simulink model "RC_protect"  (Simulink 6.4)
settings: Solver=FixedStepDiscrete  StartTime=0.0  StopTime=10.0  FixedStep=0.001  RelTol=1e-3
libraries: dsPICdrivers x4, simulink x1
CloseFcn:
  | rtwprivate ssgencode ModelCloseRequest dspic_sensorless
settings Model: DataTypeOverride=ForceOff  MinMaxOverflowLogging=ForceOff  Creator=Lubin  LastModifiedBy=lubink
settings OptimizationCC: InlineParams=on  InlineInvariantSignals=on  EnforceIntegerDowncast=off  StateBitsets=on  DataBitsets=on  UseTempVars=on  ZeroExternalMemoryAtStartup=off  ZeroInternalMemoryAtStartup=off  InitFltsAndDblsToZero=off  OptimizeModelRefInitCode=on  LifeSpan=1
settings DebuggingCC: MultiTaskDSMMsg=error  MultiTaskCondExecSysMsg=error
settings HardwareCC: ProdBitPerInt=16  ProdEndianess=LittleEndian  ProdWordSize=16  ProdHWDeviceType=16-bit Generic  TargetHWDeviceType=32-bit Generic
settings RTWCC: SystemTargetFile=dspic.tlc  TemplateMakefile=dspic_pic30_gcc.tmf  PostCodeGenCommand=dsPIC_Compile()  Description=Embedded Target for Microchip dsPIC (real-time)  GenerateReport=on  ProcessScript=dspic_make_rtw_hook  IncludeHyperlinkInReport=on  LaunchReport=on
settings CodeAppCC: IgnoreCustomStorageClasses=off
settings STFCustomTargetCC: TargetFcnLib=ansi_tfl_tmw.mat  GenFloatMathFcnCalls=ANSI_C  ModelReferenceCompliant=off  IncludeMdlTerminateFcn=off  CombineOutputUpdateFcns=on  SuppressErrorStatus=on  ERTCustomFileBanners=on  SupportContinuousTime=off  SupportNonInlinedSFcns=off  ModelStepFunctionPrototypeControlCompliant=on  SystemTargetFile=dspic.tlc
settings ERTTargetCC: TargetFcnLib=ansi_tfl_tmw.mat  GenFloatMathFcnCalls=ANSI_C  ModelReferenceCompliant=off  ParMdlRefBuildCompliant=off  CompOptLevelCompliant=off  IncludeMdlTerminateFcn=off  SuppressErrorStatus=on  ExtModeMexFile=ext_serial_win32_comm  InlinedParameterPlacement=NonHierarchical  ERTSrcFileBannerTemplate=dsPIC_code_template.cgt  ERTHdrFileBannerTemplate=dsPIC_code_template.cgt  ERTDataSrcFileTemplate=dsPIC_code_template.cgt  ERTDataHdrFileTemplate=dsPIC_code_template.cgt  ERTCustomFileTemplate=dsPIC_main.tlc
settings CustomProperty: DataType=string  Value=C:\PROGRA~1\MATLAB\R2009a\bin\win32\gmake

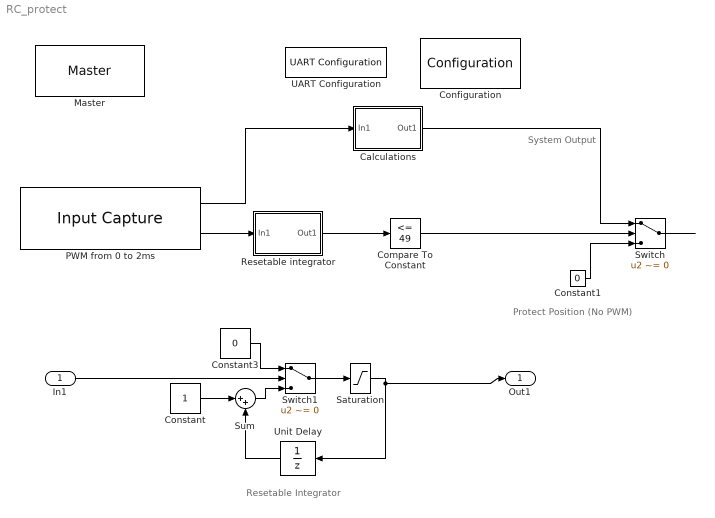
== system RC_protect ==
  note: System Output
  note: Protect Position (No PWM)
  note: Resetable Integrator
  In1 : Inport  OutDataType=sfix(16)  OutScaling=2^0
  Calculations : Subsystem
  Compare To Constant : simulink/Logic and Bit Operations/Compare To Constant  SystemSampleTime=-1  relop=<=  const=49  LogicOutDataTypeMode=boolean  ZeroCross=off
  Configuration : dsPICdrivers/Configuration  SystemSampleTime=-1  double64=off
  Constant : Constant  OutDataTypeMode=uint8  OutDataType=sfix(16)  OutScaling=2^0  SampleTime=-1
  Constant1 : Constant  Value=0  OutDataTypeMode=uint16  OutDataType=sfix(16)  OutScaling=2^0  SampleTime=-1
  Constant3 : Constant  Value=0  OutDataTypeMode=uint8  OutDataType=sfix(16)  OutScaling=2^0  SampleTime=-1
  Master : dsPICdrivers/Master  Tag=dsPIC_MASTER  Priority=1  TimeStepType=Timer1  picType=30f2010  fcy=10e6  Quartz_33f=5e6  PLLActive_33f=off  fcyDesired_33f=0  tmr1="[1  9999  0]"  tmr1Info="Time Step : 0.001  ;   Error : 0%  PR1=9999"  tmr2345="[1  0]"  tmr2345cfg=[-1 -1]  IOautoConf=on  typePort="[ 0  0  0  0  0  0  0  0  0  0  0  0  0  0  0  0  0  0  0  0  0  0  0  0  0  0  0  0  0  0  0  0  0  0  0  0  0  0  0  0  0  0  0  0  0  0  0  0  6  0  0  0  0  0  0  0  0  0  0  0  0  0  0  0  0  0  0  0  0  0  0  0  0  0  0  0  0  0  0  0  0  0  4  0  0  0  0  0  0  0  0  0  0  0  0  0  0  0  0  0  0  0  0  0  0  0  0  0  0  0  0  0 ]"  TRIS="[ 65535  65535  65535  65535  65535  65535  65535 ]"  ADPCFG=0  MasterBusyPort=None  MasterOverloadPort=None  FOSC=XT_PLL4  ClockSwitchMonitor=Both disabled  TempProtection_33f=TEMP_ON  FPBOR=BORV_20  PWRT=PWRT_16  MCLR=MCLR_DIS  PowerSave=off  OverrideFcy=off  NewFcy=1e6  PR2345="[65535  65535]"
  PWM from 0 to 2ms : dsPICdrivers/Peripheral I//O/Input Capture  Tag=dsPIC_PWM_IC  Priority=5  IntPriority=3  Channel="[1  ]"  Channel_UP_Down_Periode=[1]  MaxChannel=[0.001]  SafeMarge=[10]  MaxName=' IC1max '  Precision=[13.425]  Timer=[2]  ChangeDetected=[2]  ChangeDetectedPortRef=3  SampleTime=-1  Status=OK
  Resetable integrator : Subsystem
  Saturation : Saturate  UpperLimit=50  LowerLimit=0
  Sum : Sum  Inputs=|++  OutDataType=sfix(16)  OutScaling=2^0
  Switch : Switch  Criteria=u2 ~= 0
  Switch1 : Switch  Criteria=u2 ~= 0
  UART Configuration : dsPICdrivers/Serial PORT/UART Configuration  Tag=dsPIC_config_UART  Priority=2  UART=1  proposed_BAUD=57600  ALT_TX_RX=off  InterruptTxWhen=When Transmit Buffer is empty  TXInterruptPri=1  TxBufferSize=32  TXEN=off  InterruptRxWhen=When Receive Buffer is full (contain 4 characters)  RXInterruptPri=1  RxBufferSize=32  BAUD=57600  UxBRG=10  Info="UxBRG = 10   ||  Real Baud : 56818   ||  % error : -1.3573  ||  max 0.39773 Bytes / Step"  RealBaud=0
  Unit Delay : UnitDelay  Orientation=left  SampleTime=-1
  Out1 : Outport  OutDataType=sfix(16)  OutScaling=2^0
  wires:
  PWM from 0 to 2ms/2 -> Resetable integrator/1(In1)
  Constant1/1 -> Switch/3
  Resetable integrator/1(Out1) -> Compare To Constant/1
  Switch/1 -> ?
  Compare To Constant/1 -> Switch/2
  Constant/1 -> Sum/1
  Unit Delay/1 -> Sum/2
  Sum/1 -> Switch1/3
  Constant3/1 -> Switch1/1
  In1/1 -> Switch1/2
  Switch1/1 -> Saturation/1
  Saturation/1 -> Out1/1, Unit Delay/1
  Calculations/1(Out1) -> Switch/1
  PWM from 0 to 2ms/1 -> Calculations/1(In1)

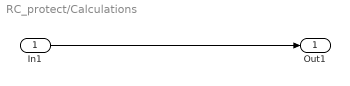
== system RC_protect/Calculations ==
  In1 : Inport  OutDataType=sfix(16)  OutScaling=2^0
  Out1 : Outport  OutDataType=sfix(16)  OutScaling=2^0
  wires:
  In1/1 -> Out1/1

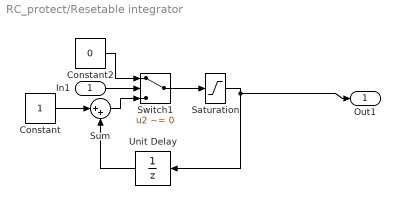
== system RC_protect/Resetable integrator ==
  In1 : Inport  OutDataType=sfix(16)  OutScaling=2^0
  Constant : Constant  OutDataTypeMode=uint8  OutDataType=sfix(16)  OutScaling=2^0  SampleTime=-1
  Constant2 : Constant  Value=0  OutDataTypeMode=uint8  OutDataType=sfix(16)  OutScaling=2^0  SampleTime=-1
  Saturation : Saturate  UpperLimit=50  LowerLimit=0
  Sum : Sum  Inputs=|++  OutDataType=sfix(16)  OutScaling=2^0
  Switch1 : Switch  Criteria=u2 ~= 0
  Unit Delay : UnitDelay  Orientation=left  SampleTime=-1
  Out1 : Outport  OutDataType=sfix(16)  OutScaling=2^0
  wires:
  Constant/1 -> Sum/1
  Unit Delay/1 -> Sum/2
  Sum/1 -> Switch1/3
  Constant2/1 -> Switch1/1
  In1/1 -> Switch1/2
  Switch1/1 -> Saturation/1
  Saturation/1 -> Unit Delay/1, Out1/1
